simulink model "flightControlSystem"  (R2026a)
settings: Solver=ode3  StartTime=0  StopTime=TFinal  FixedStep=Ts  EnableMultiTasking=on
undefined symbols (not defined in the file): codertarget, Controller, DiscIntNeverNeededParam, Discrete, Estimator, g, gray, init, Sensors, Time, Ts, var_acc_angle_N, var_bias_gyr_N, var_gyro_p_N, Vehicle
libraries: simulink x39, slpidlib x4, ctrlSharedLib x4, sharedtransform x3, parrotlib x1
(part 2 of 2)

== system flightControlSystem/Control System/Crash Predictor Flags/Normal condition ==
  Action Port : ActionPort  ActionPortLabel=else
  Constant : Constant  Value=0  OutDataTypeStr=uint8
  Out1 : Outport  VectorParamsAs1DForOutWhenUnconnected=off
  wires:
  Constant/1 -> Out1/1

== system flightControlSystem/Control System/Crash Predictor Flags/Ultrasound improper ==
  Action Port : ActionPort  ActionPortLabel=elseif(u4>0)
  Constant : Constant  Value=0  OutDataTypeStr=uint8
  Out1 : Outport  VectorParamsAs1DForOutWhenUnconnected=off
  wires:
  Constant/1 -> Out1/1

== system flightControlSystem/Control System/Crash Predictor Flags/estimator//Optical flow error ==
  Action Port : ActionPort  ActionPortLabel=elseif(u2 > 0)
  Constant : Constant  Value=99  OutDataTypeStr=uint8
  Out1 : Outport  VectorParamsAs1DForOutWhenUnconnected=off
  wires:
  Constant/1 -> Out1/1

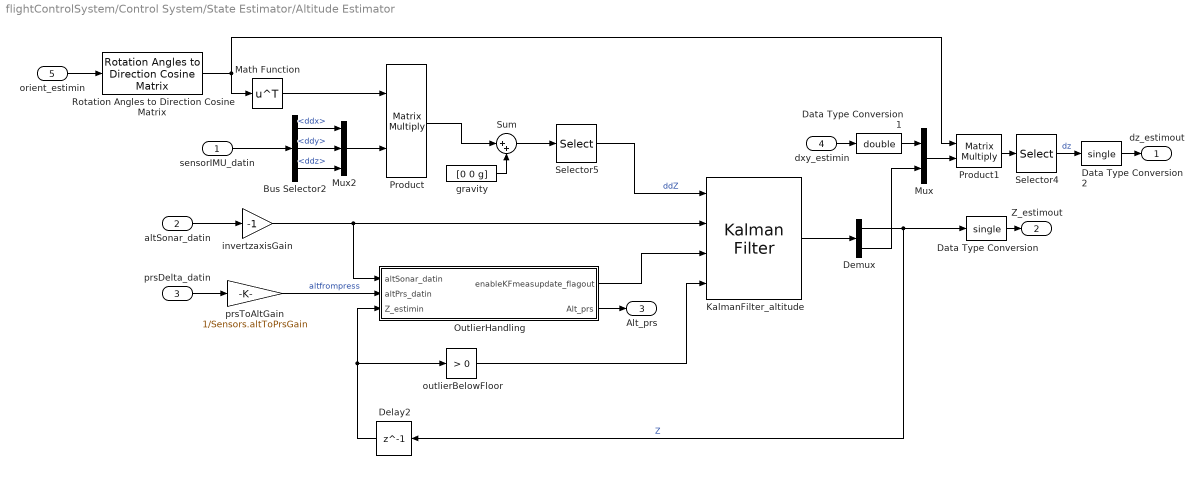
== system flightControlSystem/Control System/State Estimator/Altitude Estimator ==
  sensorIMU_datin : Inport
  altSonar_datin : Inport  Port=2
  prsDelta_datin : Inport  Port=3
  dxy_estimin : Inport  Port=4
  orient_estimin : Inport  Port=5
  Bus Selector2 : BusSelector  OutputSignals=ddx,ddy,ddz
  Data Type Conversion : DataTypeConversion  OutDataTypeStr=single  RndMeth=Floor
  Data Type Conversion1 : DataTypeConversion  OutDataTypeStr=double  RndMeth=Floor
  Data Type Conversion2 : DataTypeConversion  OutDataTypeStr=single  RndMeth=Floor
  Delay2 : Delay  DelayLength=1  InitialCondition=0
  Demux : Demux  Outputs=2
  KalmanFilter_altitude : ctrlSharedLib/Kalman Filter  TimeDomain=Discrete-Time  UseCurrentEstimator=on  ModelSource=Individual A, B, C, D matrices  ModelSourceVariable=sys  A=[1 Ts; 0 1]  B=[0;Ts]  C=[1 0]  D=[0]  NumberOfStates=2  NumberOfInputs=2  NumberOfOutputs=2  Ts=-1  InitialEstimateSource=Dialog  X0=[init.posNED(3) 0]  P0=10  UseK=off  UseGH=on  G=Estimator.alt.kf.G  TimeInvariantG=on  H=Estimator.alt.kf.H  TimeInvariantH=on  NumberOfProcessNoiseInputs=2  Q=Estimator.alt.kf.Q  TimeInvariantQ=on  R=Estimator.alt.kf.R  TimeInvariantR=on  N=Estimator.alt.kf.N  TimeInvariantN=on  AddInputPort=on  AddEnablePort=on  ExternalReset=Level hold  OutputEstimatedY=off  OutputP=off
  Math Function : Math  Operator=transpose  SignedPower=on
  Mux : Mux  Inputs=2
  Mux2 : Mux  Inputs=3
  OutlierHandling : Subsystem
  Product : Product  Multiplication=Matrix(*)
  Product1 : Product  Multiplication=Matrix(*)
  Rotation Angles to Direction Cosine Matrix : sharedtransform/Rotation Angles to Direction Cosine Matrix  rotationOrder=ZYX  aMode=aMode
  Selector4 : Selector  InputPortWidth=3  IndexOptions=Index vector (dialog)  Indices=[3]  OutputSizes=1
  Selector5 : Selector  InputPortWidth=3  IndexOptions=Index vector (dialog)  Indices=[3]  OutputSizes=1
  Sum : Sum  Inputs=|++
  gravity : Constant  Value=[0 0 g]
  invertzaxisGain : Gain  Gain=-1  ParamDataTypeStr=single  OutDataTypeStr=double
  outlierBelowFloor : simulink/Logic and Bit Operations/Compare To Constant  relop=>  const=0  OutDataTypeStr=boolean
  prsToAltGain : Gain  Gain=1/Sensors.altToPrsGain
  dz_estimout : Outport  VectorParamsAs1DForOutWhenUnconnected=off
  Z_estimout : Outport  Port=2  VectorParamsAs1DForOutWhenUnconnected=off
  Alt_prs : Outport  Port=3  VectorParamsAs1DForOutWhenUnconnected=off
  wires:
  Mux2/1 -> Product/2
  sensorIMU_datin/1 -> Bus Selector2/1
  Bus Selector2/3 -> Mux2/3  "<ddz>"
  Bus Selector2/2 -> Mux2/2  "<ddy>"
  Bus Selector2/1 -> Mux2/1  "<ddx>"
  Product1/1 -> Selector4/1
  dxy_estimin/1 -> Data Type Conversion1/1
  Delay2/1 -> OutlierHandling/3(Z_estimin), outlierBelowFloor/1
  prsToAltGain/1 -> OutlierHandling/2(altPrs_datin)  "altfrompress"
  prsDelta_datin/1 -> prsToAltGain/1
  outlierBelowFloor/1 -> KalmanFilter_altitude/4
  Demux/2 -> Mux/2
  Selector4/1 -> Data Type Conversion2/1  "dz"
  Demux/1 -> Data Type Conversion/1, Delay2/1  "Z"
  Selector5/1 -> KalmanFilter_altitude/1  "ddZ"
  Mux/1 -> Product1/2
  KalmanFilter_altitude/1 -> Demux/1
  Sum/1 -> Selector5/1
  gravity/1 -> Sum/2
  Product/1 -> Sum/1
  altSonar_datin/1 -> invertzaxisGain/1
  orient_estimin/1 -> Rotation Angles to Direction Cosine Matrix/1
  Data Type Conversion/1 -> Z_estimout/1
  Data Type Conversion1/1 -> Mux/1
  Math Function/1 -> Product/1
  invertzaxisGain/1 -> KalmanFilter_altitude/2, OutlierHandling/1(altSonar_datin)
  Data Type Conversion2/1 -> dz_estimout/1
  OutlierHandling/1(enableKFmeasupdate_flagout) -> KalmanFilter_altitude/3
  Rotation Angles to Direction Cosine Matrix/1 -> Math Function/1, Product1/1
  OutlierHandling/2(Alt_prs) -> Alt_prs/1

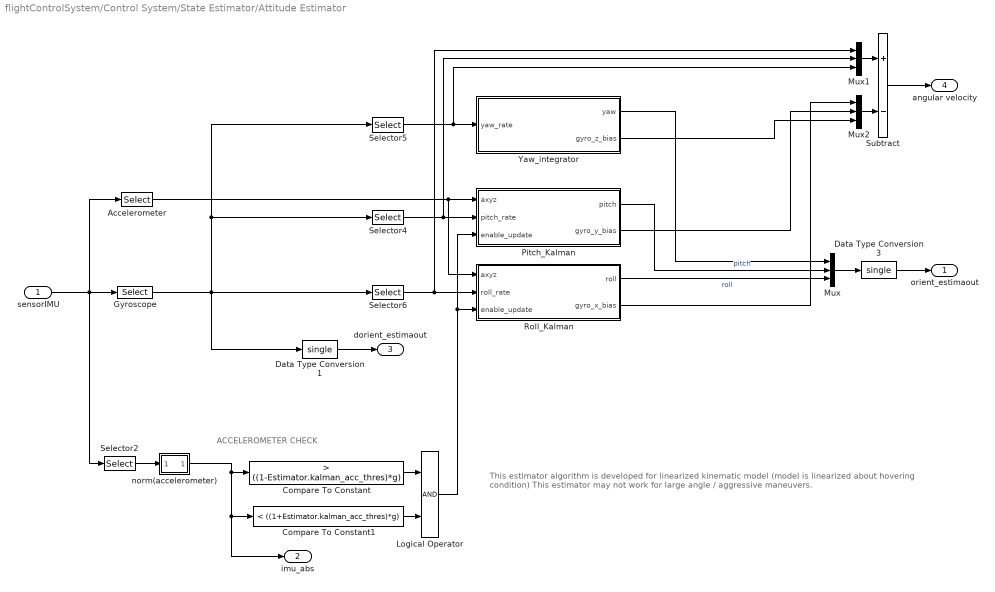
== system flightControlSystem/Control System/State Estimator/Attitude Estimator ==
  note: ACCELEROMETER CHECK
  note: This estimator algorithm is developed for linearized kinematic model (model is linearized about hovering condition)
      | This estimator may not work for large angle / aggressive maneuvers.
  sensorIMU : Inport  OutDataTypeStr=single
  Accelerometer : Selector  InputPortWidth=6  IndexOptions=Index vector (dialog)  Indices=[1 2 3]  OutputSizes=1
  Compare To Constant : simulink/Logic and Bit Operations/Compare To Constant  relop=>  const=((1-Estimator.kalman_acc_thres)*g)  OutDataTypeStr=boolean
  Compare To Constant1 : simulink/Logic and Bit Operations/Compare To Constant  relop=<  const=((1+Estimator.kalman_acc_thres)*g)  OutDataTypeStr=boolean
  Data Type Conversion1 : DataTypeConversion  OutDataTypeStr=single  SaturateOnIntegerOverflow=off  RndMeth=Floor
  Data Type Conversion3 : DataTypeConversion  OutDataTypeStr=single  SaturateOnIntegerOverflow=off  RndMeth=Floor
  Gyroscope : Selector  InputPortWidth=6  IndexOptions=Index vector (dialog)  Indices=[4 5 6]  OutputSizes=1
  Logical Operator : Logic  AllPortsSameDT=off  OutDataTypeStr=fixdt(1,16)
  Mux : Mux  Inputs=3
  Mux1 : Mux  Inputs=3
  Mux2 : Mux  Inputs=3
  Pitch_Kalman : Subsystem
  Roll_Kalman : Subsystem
  Selector2 : Selector  InputPortWidth=6  IndexOptions=Index vector (dialog)  Indices=[1 2 3]  OutputSizes=1
  Selector4 : Selector  InputPortWidth=3  IndexOptions=Index vector (dialog)  Indices=[2]  OutputSizes=1
  Selector5 : Selector  InputPortWidth=3  IndexOptions=Index vector (dialog)  Indices=[3]  OutputSizes=1
  Selector6 : Selector  InputPortWidth=3  IndexOptions=Index vector (dialog)  Indices=[1]  OutputSizes=1
  Subtract : Sum  Inputs=+-
  Yaw_integrator : Subsystem
  norm(accelerometer) : Subsystem
  orient_estimaout : Outport  VectorParamsAs1DForOutWhenUnconnected=off
  imu_abs : Outport  Port=2  OutDataTypeStr=single  VectorParamsAs1DForOutWhenUnconnected=off
  dorient_estimaout : Outport  Port=3  VectorParamsAs1DForOutWhenUnconnected=off
  angular velocity : Outport  Port=4  VectorParamsAs1DForOutWhenUnconnected=off
  wires:
  sensorIMU/1 -> Selector2/1, Accelerometer/1, Gyroscope/1
  Compare To Constant/1 -> Logical Operator/1
  Compare To Constant1/1 -> Logical Operator/2
  Mux/1 -> Data Type Conversion3/1
  Gyroscope/1 -> Data Type Conversion1/1, Selector5/1, Selector4/1, Selector6/1
  Data Type Conversion3/1 -> orient_estimaout/1
  Data Type Conversion1/1 -> dorient_estimaout/1
  Accelerometer/1 -> Roll_Kalman/1(axyz), Pitch_Kalman/1(axyz)
  Selector4/1 -> Mux1/2, Pitch_Kalman/2(pitch_rate)
  Selector5/1 -> Mux1/3, Yaw_integrator/1(yaw_rate)
  Selector6/1 -> Mux1/1, Roll_Kalman/2(roll_rate)
  Yaw_integrator/1(yaw) -> Mux/1
  Pitch_Kalman/1(pitch) -> Mux/2  "pitch"
  Roll_Kalman/1(roll) -> Mux/3  "roll"
  Logical Operator/1 -> Roll_Kalman/3(enable_update), Pitch_Kalman/3(enable_update)
  Mux1/1 -> Subtract/1
  Subtract/1 -> angular velocity/1
  Roll_Kalman/2(gyro_x_bias) -> Mux2/1
  Pitch_Kalman/2(gyro_y_bias) -> Mux2/2
  Yaw_integrator/2(gyro_z_bias) -> Mux2/3
  Mux2/1 -> Subtract/2
  norm(accelerometer)/1(Out1) -> imu_abs/1, Compare To Constant1/1, Compare To Constant/1
  Selector2/1 -> norm(accelerometer)/1(In1)

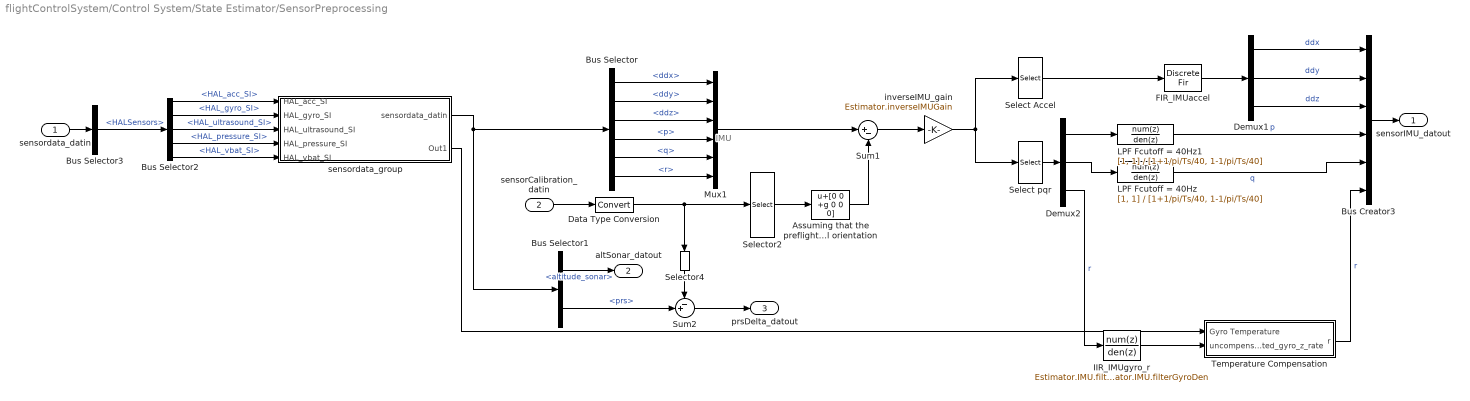
== system flightControlSystem/Control System/State Estimator/SensorPreprocessing ==
  note: IMU
  sensordata_datin : Inport
  sensorCalibration_datin : Inport  Port=2
  Assuming that the preflight calibration was done at level orientation : Bias  Bias=[0 0 +g 0 0 0]  SaturateOnIntegerOverflow=off
  Bus Creator3 : BusCreator  Inputs=6
  Bus Selector : BusSelector  OutputSignals=ddx,ddy,ddz,p,q,r
  Bus Selector1 : BusSelector  OutputSignals=altitude_sonar,prs
  Bus Selector2 : BusSelector  OutputSignals=HAL_acc_SI,HAL_gyro_SI,HAL_ultrasound_SI,HAL_pressure_SI,HAL_vbat_SI
  Bus Selector3 : BusSelector  OutputSignals=HALSensors
  Data Type Conversion : DataTypeConversion  SaturateOnIntegerOverflow=off  RndMeth=Floor
  Demux1 : Demux  Outputs=3
  Demux2 : Demux  Outputs=3
  FIR_IMUaccel : DiscreteFir  Coefficients=Estimator.IMU.filterAccel.Coefficients
  IIR_IMUgyro_r : DiscreteFilter  Numerator=Estimator.IMU.filterGyroNum  Denominator=Estimator.IMU.filterGyroDen
  LPF Fcutoff = 40Hz : DiscreteTransferFcn  Numerator=[1, 1]  Denominator=[1+1/pi/Ts/40, 1-1/pi/Ts/40]
  LPF Fcutoff = 40Hz1 : DiscreteTransferFcn  Numerator=[1, 1]  Denominator=[1+1/pi/Ts/40, 1-1/pi/Ts/40]
  Mux1 : Mux  Inputs=6
  Select Accel : Selector  InputPortWidth=6  IndexOptions=Index vector (dialog)  Indices=[1 2 3]  OutputSizes=1
  Select pqr : Selector  InputPortWidth=6  IndexOptions=Index vector (dialog)  Indices=[4 5 6]  OutputSizes=1
  Selector2 : Selector  InputPortWidth=8  IndexOptions=Index vector (dialog)  Indices=[1:6]  OutputSizes=1
  Selector4 : Selector  InputPortWidth=8  IndexOptions=Index vector (dialog)  Indices=[7]  OutputSizes=1
  Sum1 : Sum  Inputs=|+-
  Sum2 : Sum  Inputs=-+|
  Temperature Compensation : Subsystem
  inverseIMU_gain : Gain  Gain=Estimator.inverseIMUGain  ParamDataTypeStr=single  OutDataTypeStr=single
  sensordata_group : Subsystem
  sensorIMU_datout : Outport  VectorParamsAs1DForOutWhenUnconnected=off
  altSonar_datout : Outport  Port=2  VectorParamsAs1DForOutWhenUnconnected=off
  prsDelta_datout : Outport  Port=3  VectorParamsAs1DForOutWhenUnconnected=off
  wires:
  Select pqr/1 -> Demux2/1
  Assuming that the preflight calibration was done at level orientation/1 -> Sum1/2
  Mux1/1 -> Sum1/1
  Sum2/1 -> prsDelta_datout/1
  Bus Selector1/2 -> Sum2/2  "<prs>"
  Selector4/1 -> Sum2/1
  Bus Selector1/1 -> altSonar_datout/1  "<altitude_sonar>"
  Bus Selector/6 -> Mux1/6  "<r>"
  Bus Selector/5 -> Mux1/5  "<q>"
  Bus Selector/4 -> Mux1/4  "<p>"
  Bus Selector/3 -> Mux1/3  "<ddz>"
  Bus Selector/2 -> Mux1/2  "<ddy>"
  Bus Selector/1 -> Mux1/1  "<ddx>"
  sensorCalibration_datin/1 -> Data Type Conversion/1
  Demux2/3 -> IIR_IMUgyro_r/1  "r"
  FIR_IMUaccel/1 -> Demux1/1
  Select Accel/1 -> FIR_IMUaccel/1
  inverseIMU_gain/1 -> Select Accel/1, Select pqr/1
  Demux2/2 -> LPF Fcutoff = 40Hz/1
  Demux2/1 -> LPF Fcutoff = 40Hz1/1
  Selector2/1 -> Assuming that the preflight calibration was done at level orientation/1
  Sum1/1 -> inverseIMU_gain/1
  Demux1/3 -> Bus Creator3/3  "ddz"
  Demux1/2 -> Bus Creator3/2  "ddy"
  Demux1/1 -> Bus Creator3/1  "ddx"
  Bus Creator3/1 -> sensorIMU_datout/1
  Data Type Conversion/1 -> Selector2/1, Selector4/1
  Bus Selector2/2 -> sensordata_group/2(HAL_gyro_SI)  "<HAL_gyro_SI>"
  Bus Selector2/4 -> sensordata_group/4(HAL_pressure_SI)  "<HAL_pressure_SI>"
  Bus Selector2/5 -> sensordata_group/5(HAL_vbat_SI)  "<HAL_vbat_SI>"
  Bus Selector2/3 -> sensordata_group/3(HAL_ultrasound_SI)  "<HAL_ultrasound_SI>"
  Bus Selector3/1 -> Bus Selector2/1  "<HALSensors>"
  sensordata_group/1(sensordata_datin) -> Bus Selector1/1, Bus Selector/1
  sensordata_datin/1 -> Bus Selector3/1
  Bus Selector2/1 -> sensordata_group/1(HAL_acc_SI)  "<HAL_acc_SI>"
  LPF Fcutoff = 40Hz1/1 -> Bus Creator3/4  "p"
  LPF Fcutoff = 40Hz/1 -> Bus Creator3/5  "q"
  sensordata_group/2(Out1) -> Temperature Compensation/1(Gyro Temperature)
  IIR_IMUgyro_r/1 -> Temperature Compensation/2(uncompensated_gyro_z_rate)
  Temperature Compensation/1(r) -> Bus Creator3/6  "r"

== system flightControlSystem/Control System/State Estimator/XY Position Estimator ==
  opticalFlow_datin : Inport
  controlModePosVSOrient_flagin : Inport  Port=2
  sensorIMU_datin : Inport  Port=3
  Z_estimin : Inport  Port=4
  dz_estimin : Inport  Port=5
  orient_estimin : Inport  Port=6
  Angular velocity : Inport  Port=7
  EstimatorVelocity : Subsystem
  EstimatorXYPosition : Subsystem
  XY_estimout : Outport  VectorParamsAs1DForOutWhenUnconnected=off
  dxy_estimout : Outport  Port=2  VectorParamsAs1DForOutWhenUnconnected=off
  wires:
  EstimatorXYPosition/1(XY_estimout) -> XY_estimout/1
  dz_estimin/1 -> EstimatorXYPosition/4(dz_estimin)
  controlModePosVSOrient_flagin/1 -> EstimatorXYPosition/3(controlModePosVSOrient_flagin)
  Z_estimin/1 -> EstimatorVelocity/2(Z_estimin)
  sensorIMU_datin/1 -> EstimatorVelocity/3(sensorIMU_datin)
  opticalFlow_datin/1 -> EstimatorVelocity/1(opticalFlow_datin)
  EstimatorVelocity/1(dxy_estimout) -> dxy_estimout/1, EstimatorXYPosition/1(dxy_estimin)
  orient_estimin/1 -> EstimatorXYPosition/2(orient_estimin), EstimatorVelocity/4(orient_estimin)
  Angular velocity/1 -> EstimatorVelocity/5(angular velocity)

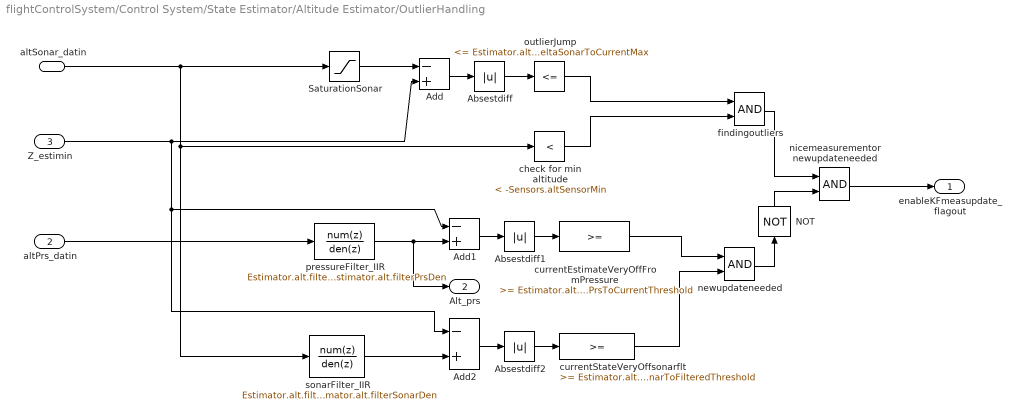
== system flightControlSystem/Control System/State Estimator/Altitude Estimator/OutlierHandling ==
  altSonar_datin : Inport
  altPrs_datin : Inport  Port=2
  Z_estimin : Inport  Port=3
  Absestdiff : Abs  SaturateOnIntegerOverflow=off
  Absestdiff1 : Abs  SaturateOnIntegerOverflow=off
  Absestdiff2 : Abs  SaturateOnIntegerOverflow=off
  Add : Sum  Inputs=-+
  Add1 : Sum  Inputs=-+
  Add2 : Sum  Inputs=-+
  NOT : Logic  Operator=NOT  IconShape=distinctive  AllPortsSameDT=off  OutDataTypeStr=boolean
  SaturationSonar : Saturate  UpperLimit=-Sensors.altSensorMin  LowerLimit=-inf
  check for min altitude : simulink/Logic and Bit Operations/Compare To Constant  relop=<  const=-Sensors.altSensorMin  OutDataTypeStr=boolean
  currentEstimateVeryOffFromPressure : simulink/Logic and Bit Operations/Compare To Constant  relop=>=  const=Estimator.alt.deltaPrsToCurrentThreshold  OutDataTypeStr=boolean
  currentStateVeryOffsonarflt : simulink/Logic and Bit Operations/Compare To Constant  relop=>=  const=Estimator.alt.deltaSonarToFilteredThreshold  OutDataTypeStr=boolean
  findingoutliers : Logic  AllPortsSameDT=off  OutDataTypeStr=boolean
  newupdateneeded : Logic  AllPortsSameDT=off  OutDataTypeStr=boolean
  nicemeasurementor newupdateneeded : Logic  AllPortsSameDT=off  OutDataTypeStr=boolean
  outlierJump : simulink/Logic and Bit Operations/Compare To Constant  relop=<=  const=Estimator.alt.deltaSonarToCurrentMax  OutDataTypeStr=boolean
  pressureFilter_IIR : DiscreteFilter  Numerator=Estimator.alt.filterPrsNum  Denominator=Estimator.alt.filterPrsDen
  sonarFilter_IIR : DiscreteFilter  Numerator=Estimator.alt.filterSonarNum  Denominator=Estimator.alt.filterSonarDen
  enableKFmeasupdate_flagout : Outport  VectorParamsAs1DForOutWhenUnconnected=off
  Alt_prs : Outport  Port=2  VectorParamsAs1DForOutWhenUnconnected=off
  wires:
  Add1/1 -> Absestdiff1/1
  nicemeasurementor newupdateneeded/1 -> enableKFmeasupdate_flagout/1
  findingoutliers/1 -> nicemeasurementor newupdateneeded/1
  check for min altitude/1 -> findingoutliers/2
  outlierJump/1 -> findingoutliers/1
  SaturationSonar/1 -> Add/1
  Absestdiff/1 -> outlierJump/1
  Add/1 -> Absestdiff/1
  newupdateneeded/1 -> NOT/1
  Absestdiff2/1 -> currentStateVeryOffsonarflt/1
  altSonar_datin/1 -> SaturationSonar/1, sonarFilter_IIR/1, check for min altitude/1
  currentEstimateVeryOffFromPressure/1 -> newupdateneeded/1
  Z_estimin/1 -> Add1/1, Add2/1, Add/2
  Add2/1 -> Absestdiff2/1
  currentStateVeryOffsonarflt/1 -> newupdateneeded/2
  pressureFilter_IIR/1 -> Alt_prs/1, Add1/2
  altPrs_datin/1 -> pressureFilter_IIR/1
  sonarFilter_IIR/1 -> Add2/2
  Absestdiff1/1 -> currentEstimateVeryOffFromPressure/1
  NOT/1 -> nicemeasurementor newupdateneeded/2

== system flightControlSystem/Control System/State Estimator/Attitude Estimator/Pitch_Kalman ==
  note: Gyroscope's bias is susceptible to factors like "temperature" and "Gyro bias stability" and it
      | can vary during the flight. It is therefore estimated using this Kalman filter making use of Accelerometer data
  note: Linear Kalman filter is used for the Pitch and Roll estimation.
      | The states are the corresponding Euler angle and Angular rate bias respectively
  axyz : Inport
  pitch_rate : Inport  Port=2
  enable_update : Inport  Port=3
  Demux : Demux  Outputs=2
  Gain2 : Gain  Gain=1/g
  Kalman Filter : ctrlSharedLib/Kalman Filter  TimeDomain=Discrete-Time  UseCurrentEstimator=on  ModelSource=Individual A, B, C, D matrices  ModelSourceVariable=ss(0.95,1,1,0,1)  A=[1 -Ts;0 1]  B=[Ts;0]  C=[1 0]  D=0  NumberOfStates=1  NumberOfInputs=1  NumberOfOutputs=1  Ts=Ts  InitialEstimateSource=Dialog  X0=0  P0=10  UseK=off  UseGH=off  G=1  TimeInvariantG=on  H=0  TimeInvariantH=on  NumberOfProcessNoiseInputs=1  Q=[var_gyro_p_N,0;0,var_bias_gyr_N]  TimeInvariantQ=on  R=var_acc_angle_N  TimeInvariantR=on  N=0  TimeInvariantN=on  AddInputPort=on  AddEnablePort=on  OutputEstimatedY=off  OutputP=off
  Selector1 : Selector  InputPortWidth=3  IndexOptions=Index vector (dialog)  Indices=[1]  OutputSizes=1
  Trigonometric Function1 : Trigonometry  Operator=asin
  single : DataTypeConversion  OutDataTypeStr=single  SaturateOnIntegerOverflow=off  RndMeth=Floor
  single1 : DataTypeConversion  OutDataTypeStr=single  SaturateOnIntegerOverflow=off  RndMeth=Floor
  pitch : Outport
  gyro_y_bias : Outport  Port=2
  wires:
  Kalman Filter/1 -> Demux/1
  Demux/1 -> single1/1
  Gain2/1 -> Trigonometric Function1/1
  Trigonometric Function1/1 -> Kalman Filter/2
  Selector1/1 -> Gain2/1
  axyz/1 -> Selector1/1
  pitch_rate/1 -> Kalman Filter/1
  enable_update/1 -> Kalman Filter/3
  Demux/2 -> single/1
  single/1 -> gyro_y_bias/1
  single1/1 -> pitch/1

== system flightControlSystem/Control System/State Estimator/Attitude Estimator/Roll_Kalman ==
  note: Linear Kalman filter is used for the Pitch and Roll estimation.
      | The states are the corresponding Euler angle and Angular rate bias respectively
  note: Gyroscope's bias is susceptible to factors like "temperature" and "Gyro bias stability" and it
      | can vary during the flight. It is therefore estimated using the Kalman filter making use of accelerometer data
  axyz : Inport
  roll_rate : Inport  Port=2
  enable_update : Inport  Port=3
  Data Type Conversion : DataTypeConversion  SaturateOnIntegerOverflow=off  RndMeth=Floor
  Data Type Conversion1 : DataTypeConversion  SaturateOnIntegerOverflow=off  RndMeth=Floor
  Demux : Demux  Outputs=3
  Demux1 : Demux  Outputs=2
  Divide : Product  Inputs=*/
  Kalman Filter : ctrlSharedLib/Kalman Filter  TimeDomain=Discrete-Time  UseCurrentEstimator=on  ModelSource=Individual A, B, C, D matrices  ModelSourceVariable=ss(0.95,1,1,0,1)  A=[1 -Ts;0 1]  B=[Ts;0]  C=[1 0]  D=0  NumberOfStates=1  NumberOfInputs=1  NumberOfOutputs=1  Ts=Ts  InitialEstimateSource=Dialog  X0=0  P0=10  UseK=off  UseGH=off  G=1  TimeInvariantG=on  H=0  TimeInvariantH=on  NumberOfProcessNoiseInputs=1  Q=[var_gyro_p_N,0;0,var_bias_gyr_N]  TimeInvariantQ=on  R=var_acc_angle_N  TimeInvariantR=on  N=0  TimeInvariantN=on  AddInputPort=on  AddEnablePort=on  OutputEstimatedY=off  OutputP=off
  Terminator : Terminator
  Trigonometric Function : Trigonometry  Operator=atan
  roll : Outport
  gyro_x_bias : Outport  Port=2
  wires:
  Demux1/1 -> Data Type Conversion1/1
  Kalman Filter/1 -> Demux1/1
  roll_rate/1 -> Kalman Filter/1
  Divide/1 -> Trigonometric Function/1
  Demux/2 -> Divide/1
  axyz/1 -> Demux/1
  Demux/3 -> Divide/2
  Trigonometric Function/1 -> Kalman Filter/2
  enable_update/1 -> Kalman Filter/3
  Demux1/2 -> Data Type Conversion/1
  Data Type Conversion/1 -> gyro_x_bias/1
  Data Type Conversion1/1 -> roll/1
  Demux/1 -> Terminator/1

== system flightControlSystem/Control System/State Estimator/Attitude Estimator/Yaw_integrator ==
  note: Yaw angle is not constrained between -180 to 180 degrees
  note: Currently yaw angle is obtained solely by integrating the gyroscope output.
      | This yaw estimate can drift with time.
  yaw_rate : Inport
  Constant : Constant  Value=0  OutDataTypeStr=single
  Discrete-Time Integrator : DiscreteIntegrator  SampleTime=-1  ICPrevOutput=DiscIntNeverNeededParam  ICPrevScaledInput=DiscIntNeverNeededParam
  yaw : Outport
  gyro_z_bias : Outport  Port=2
  wires:
  yaw_rate/1 -> Discrete-Time Integrator/1
  Discrete-Time Integrator/1 -> yaw/1
  Constant/1 -> gyro_z_bias/1

== system flightControlSystem/Control System/State Estimator/Attitude Estimator/norm(accelerometer) ==
  In1 : Inport
  Constant : Constant  Value=2  OutDataTypeStr=single
  Data Type Conversion2 : DataTypeConversion  OutDataTypeStr=single  SaturateOnIntegerOverflow=off  RndMeth=Floor
  Math Function : Math  Operator=pow  SignedPower=on
  Sqrt : Sqrt
  Sum of Elements : Sum  Inputs=+
  Out1 : Outport
  wires:
  Sum of Elements/1 -> Sqrt/1
  Math Function/1 -> Sum of Elements/1
  Data Type Conversion2/1 -> Math Function/1
  In1/1 -> Data Type Conversion2/1
  Constant/1 -> Math Function/2
  Sqrt/1 -> Out1/1

== system flightControlSystem/Control System/State Estimator/SensorPreprocessing/Temperature Compensation ==
  note: Gyroscope's bias is affected by temperature.This won't be a problem for Pitch and Roll angle estimation as the actual gyroscope bias in the Pitch and Roll axis are estimated during the flight. However the yaw orientation is obtained by integrating the gyroscope output and it may drift with time. Even the preflight calibration which is done cannot compensate for this problem as the gyro bis varies during the flight.
  Gyro Temperature : Inport
  uncompensated_gyro_z_rate : Inport  Port=2
  Compare To Constant : simulink/Logic and Bit Operations/Compare To Constant  relop===  const=1  OutDataTypeStr=boolean
  Constant : Constant  Value=0
  Counter Free-Running : simulink/Sources/Counter Free-Running  NumBits=32  tsamp=0.005
  Data Type Conversion1 : DataTypeConversion  SaturateOnIntegerOverflow=off  RndMeth=Floor
  Disable temperature compensation : ManualSwitch
  Gain : Gain  Gain=0.00228
  Subtract : Sum  Inputs=+-
  Subtract1 : Sum  Inputs=+-
  Triggered Subsystem : Subsystem  TreatAsAtomicUnit=on
  r : Outport
  wires:
  Gain/1 -> Disable temperature compensation/1
  Disable temperature compensation/1 -> Data Type Conversion1/1
  Gyro Temperature/1 -> Subtract/1, Triggered Subsystem/1(In1)
  Triggered Subsystem/1(Out1) -> Subtract/2  "Initial temperature"
  Compare To Constant/1 -> Triggered Subsystem/Trigger
  Constant/1 -> Disable temperature compensation/2
  Subtract/1 -> Gain/1
  Data Type Conversion1/1 -> Subtract1/2
  Counter Free-Running/1 -> Compare To Constant/1
  uncompensated_gyro_z_rate/1 -> Subtract1/1
  Subtract1/1 -> r/1  "r"

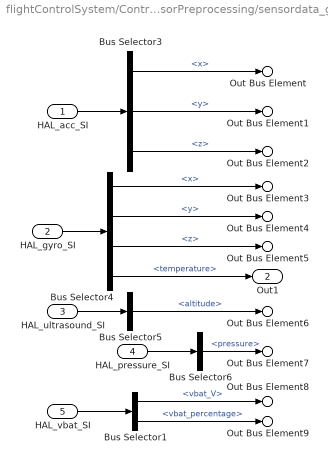
== system flightControlSystem/Control System/State Estimator/SensorPreprocessing/sensordata_group ==
  HAL_acc_SI : Inport  OutDataTypeStr=Bus: HAL_acc_SI_t
  HAL_gyro_SI : Inport  Port=2  OutDataTypeStr=Bus: HAL_gyro_SI_t
  HAL_ultrasound_SI : Inport  Port=3  OutDataTypeStr=Bus: HAL_ultrasound_SI_t
  HAL_pressure_SI : Inport  Port=4  OutDataTypeStr=Bus: HAL_pressure_SI_t
  HAL_vbat_SI : Inport  Port=5  OutDataTypeStr=Bus: HAL_vbat_SI_t
  Bus Selector1 : BusSelector  OutputSignals=vbat_V,vbat_percentage
  Bus Selector3 : BusSelector  OutputSignals=x,y,z
  Bus Selector4 : BusSelector  OutputSignals=x,y,z,temperature
  Bus Selector5 : BusSelector  OutputSignals=altitude
  Bus Selector6 : BusSelector  OutputSignals=pressure
  Out Bus Element : Outport  VectorParamsAs1DForOutWhenUnconnected=off  PortName=sensordata_datin  Element=ddx
  Out Bus Element1 : Outport  VectorParamsAs1DForOutWhenUnconnected=off  PortName=sensordata_datin  Element=ddy
  Out Bus Element2 : Outport  VectorParamsAs1DForOutWhenUnconnected=off  PortName=sensordata_datin  Element=ddz
  Out Bus Element3 : Outport  VectorParamsAs1DForOutWhenUnconnected=off  PortName=sensordata_datin  Element=p
  Out Bus Element4 : Outport  VectorParamsAs1DForOutWhenUnconnected=off  PortName=sensordata_datin  Element=q
  Out Bus Element5 : Outport  VectorParamsAs1DForOutWhenUnconnected=off  PortName=sensordata_datin  Element=r
  Out Bus Element6 : Outport  VectorParamsAs1DForOutWhenUnconnected=off  PortName=sensordata_datin  Element=altitude_sonar
  Out Bus Element7 : Outport  VectorParamsAs1DForOutWhenUnconnected=off  PortName=sensordata_datin  Element=prs
  Out Bus Element8 : Outport  VectorParamsAs1DForOutWhenUnconnected=off  PortName=sensordata_datin  Element=vbat_V
  Out Bus Element9 : Outport  VectorParamsAs1DForOutWhenUnconnected=off  PortName=sensordata_datin  Element=vbat_percentage
  Out1 : Outport  Port=2
  wires:
  HAL_gyro_SI/1 -> Bus Selector4/1
  HAL_acc_SI/1 -> Bus Selector3/1
  HAL_pressure_SI/1 -> Bus Selector6/1
  HAL_ultrasound_SI/1 -> Bus Selector5/1
  Bus Selector4/1 -> Out Bus Element3/1  "<x>"
  Bus Selector3/3 -> Out Bus Element2/1  "<z>"
  Bus Selector4/3 -> Out Bus Element5/1  "<z>"
  Bus Selector5/1 -> Out Bus Element6/1  "<altitude>"
  Bus Selector6/1 -> Out Bus Element7/1  "<pressure>"
  Bus Selector4/2 -> Out Bus Element4/1  "<y>"
  Bus Selector3/1 -> Out Bus Element/1  "<x>"
  Bus Selector3/2 -> Out Bus Element1/1  "<y>"
  Bus Selector1/1 -> Out Bus Element8/1  "<vbat_V>"
  HAL_vbat_SI/1 -> Bus Selector1/1
  Bus Selector1/2 -> Out Bus Element9/1  "<vbat_percentage>"
  Bus Selector4/4 -> Out1/1  "<temperature>"

== system flightControlSystem/Control System/State Estimator/XY Position Estimator/EstimatorVelocity ==
  opticalFlow_datin : Inport
  Z_estimin : Inport  Port=2  SampleTime=Ts
  sensorIMU_datin : Inport  Port=3
  orient_estimin : Inport  Port=4
  angular velocity : Inport  Port=5
  AccelerationHandling : Subsystem
  Angular velocity compensation for optical flow : Subsystem
  DataHandling : Subsystem
  Delay : Delay  DelayLength=1  InitialCondition=0
  KalmanFilter_dxdy : ctrlSharedLib/Kalman Filter  TimeDomain=Discrete-Time  UseCurrentEstimator=on  ModelSource=Individual A, B, C, D matrices  ModelSourceVariable=ss(0.95,1,1,0,1)  A=Estimator.pos.kfVelo.A  B=Estimator.pos.kfVelo.B  C=Estimator.pos.kfVelo.C  D=Estimator.pos.kfVelo.D  NumberOfStates=1  NumberOfInputs=1  NumberOfOutputs=1  Ts=-1  InitialEstimateSource=Dialog  X0=0  P0=10  UseK=off  UseGH=off  G=Estimator.pos.kfVelo.G  TimeInvariantG=on  H=Estimator.pos.kfVelo.H  TimeInvariantH=on  NumberOfProcessNoiseInputs=1  Q=Estimator.pos.kfVelo.Q  TimeInvariantQ=on  R=Estimator.pos.kfVelo.R  TimeInvariantR=on  N=Estimator.pos.kfVelo.N  TimeInvariantN=on  AddInputPort=on  AddEnablePort=on  OutputEstimatedY=off  OutputP=off
  Selector1 : Selector  InputPortWidth=4  IndexOptions=Index vector (dialog)  Indices=[1 2]  OutputSizes=1
  Z_estimin1 : InportShadow  Port=2  SampleTime=Ts
  angular velocity compensation : Sum
  xy velocity w/o angular velocity compensation : Subsystem
  dxy_estimout : Outport  VectorParamsAs1DForOutWhenUnconnected=off
  wires:
  Z_estimin/1 -> DataHandling/1(Z_estimin), AccelerationHandling/4(Z_estimin)
  KalmanFilter_dxdy/1 -> Selector1/1
  sensorIMU_datin/1 -> AccelerationHandling/2(sensorIMU_datin), DataHandling/3(sensorIMU_datin)
  orient_estimin/1 -> AccelerationHandling/3(orient_estimin), DataHandling/2(orient_estimin)
  Z_estimin1/1 -> xy velocity w/o angular velocity compensation/2(z_estimate), Angular velocity compensation for optical flow/1(z_estimate)
  AccelerationHandling/1(acceleration_world) -> KalmanFilter_dxdy/1
  angular velocity compensation/1 -> KalmanFilter_dxdy/2
  Delay/1 -> DataHandling/5(dxyOF_datin)
  Selector1/1 -> dxy_estimout/1, Delay/1
  angular velocity/1 -> Angular velocity compensation for optical flow/2(Angular velocity w/o bias)
  Angular velocity compensation for optical flow/1(angular velocity correction) -> angular velocity compensation/2
  xy velocity w/o angular velocity compensation/1(optical_flow_dx_dy) -> DataHandling/4(dxy_estimin), AccelerationHandling/1(dxy_estimin), angular velocity compensation/1
  opticalFlow_datin/1 -> xy velocity w/o angular velocity compensation/1(optical_flow)
  DataHandling/1(enable_flag) -> KalmanFilter_dxdy/3

== system flightControlSystem/Control System/State Estimator/XY Position Estimator/EstimatorXYPosition ==
  note: Switching from orientationControl to Position
      | control reset the current world position estimate
      | (happens when using no markers)
  dxy_estimin : Inport
  orient_estimin : Inport  Port=2  SampleTime=Ts
  controlModePosVSOrient_flagin : Inport  Port=3
  dz_estimin : Inport  Port=4
  Math Function : Math  Operator=transpose  SignedPower=on
  Mux2 : Mux  Inputs=2
  Product : Product  Multiplication=Matrix(*)
  Rotation Angles to Direction Cosine Matrix : sharedtransform/Rotation Angles to Direction Cosine Matrix  rotationOrder=ZYX  aMode=aMode
  SelectdXY : Selector  InputPortWidth=3  IndexOptions=Index vector (dialog)  Indices=[1 2]  OutputSizes=1
  SimplyIntegrateVelocity : DiscreteIntegrator  ExternalReset=rising  SampleTime=Ts  ICPrevOutput=DiscIntNeverNeededParam  ICPrevScaledInput=DiscIntNeverNeededParam
  XY_estimout : Outport  VectorParamsAs1DForOutWhenUnconnected=off
  wires:
  controlModePosVSOrient_flagin/1 -> SimplyIntegrateVelocity/2
  Product/1 -> SelectdXY/1
  Mux2/1 -> Product/2
  dz_estimin/1 -> Mux2/2
  SimplyIntegrateVelocity/1 -> XY_estimout/1
  dxy_estimin/1 -> Mux2/1
  orient_estimin/1 -> Rotation Angles to Direction Cosine Matrix/1
  Rotation Angles to Direction Cosine Matrix/1 -> Math Function/1
  SelectdXY/1 -> SimplyIntegrateVelocity/1
  Math Function/1 -> Product/1

== system flightControlSystem/Control System/State Estimator/SensorPreprocessing/Temperature Compensation/Triggered Subsystem ==
  In1 : Inport
  Trigger : TriggerPort  TriggerType=either  VariantControl=Variant
  Out1 : Outport
  wires:
  In1/1 -> Out1/1

== system flightControlSystem/Control System/State Estimator/XY Position Estimator/EstimatorVelocity/AccelerationHandling ==
  dxy_estimin : Inport
  sensorIMU_datin : Inport  Port=2
  orient_estimin : Inport  Port=3
  Z_estimin : Inport  Port=4
  Add : Sum  Inputs=-+
  Bus Selector1 : BusSelector  OutputSignals=ddx,ddy,ddz
  Deactivate Acceleration If OF is not used due to low altitude : simulink/Logic and Bit Operations/Compare To Constant  relop=<=  const=Estimator.pos.opticalFlowZMax  OutDataTypeStr=boolean
  Logical Operator : Logic  Operator=OR  AllPortsSameDT=off  OutDataTypeStr=boolean
  Mux6 : Mux  Inputs=3
  Product : Product  Inputs=3
  Product1 : Product  Multiplication=Matrix(*)
  Rotation Angles to Direction Cosine Matrix : sharedtransform/Rotation Angles to Direction Cosine Matrix  rotationOrder=ZYX  aMode=aMode
  SelectPlanarddxy : Selector  InputPortWidth=3  IndexOptions=Index vector (dialog)  Indices=[1 2]  OutputSizes=1
  Selector : Selector  InputPortWidth=2  IndexOptions=Index vector (dialog)  Indices=1  OutputSizes=1
  Selector1 : Selector  InputPortWidth=2  IndexOptions=Index vector (dialog)  Indices=2  OutputSizes=1
  do not use acc if optical flow never available (Note OF@60Hz but ZOH to 200!) : simulink/Logic and Bit Operations/Compare To Constant  relop=~=  const=0  OutDataTypeStr=boolean
  do not use acc if optical flow never available (Note OF@60Hz but ZOH to 200!)1 : simulink/Logic and Bit Operations/Compare To Constant  relop=~=  const=0  OutDataTypeStr=boolean
  gainaccinput1 : Gain  OutDataTypeStr=single
  gravity : Constant  Value=[0 0 -g]
  acceleration_world : Outport  OutDataTypeStr=single  VectorParamsAs1DForOutWhenUnconnected=off
  wires:
  do not use acc if optical flow never available (Note OF@60Hz but ZOH to 200!)1/1 -> Logical Operator/2
  do not use acc if optical flow never available (Note OF@60Hz but ZOH to 200!)/1 -> Logical Operator/1
  Logical Operator/1 -> Product/1
  Selector1/1 -> do not use acc if optical flow never available (Note OF@60Hz but ZOH to 200!)1/1
  Selector/1 -> do not use acc if optical flow never available (Note OF@60Hz but ZOH to 200!)/1
  dxy_estimin/1 -> Selector1/1, Selector/1
  Product/1 -> acceleration_world/1
  Deactivate Acceleration If OF is not used due to low altitude/1 -> Product/3
  Z_estimin/1 -> Deactivate Acceleration If OF is not used due to low altitude/1
  Add/1 -> SelectPlanarddxy/1
  Product1/1 -> Add/1
  gravity/1 -> Product1/2
  SelectPlanarddxy/1 -> gainaccinput1/1
  Bus Selector1/3 -> Mux6/3  "<ddz>"
  Bus Selector1/1 -> Mux6/1  "<ddx>"
  sensorIMU_datin/1 -> Bus Selector1/1
  Mux6/1 -> Add/2
  Bus Selector1/2 -> Mux6/2  "<ddy>"
  orient_estimin/1 -> Rotation Angles to Direction Cosine Matrix/1
  Rotation Angles to Direction Cosine Matrix/1 -> Product1/1
  gainaccinput1/1 -> Product/2

== system flightControlSystem/Control System/State Estimator/XY Position Estimator/EstimatorVelocity/Angular velocity compensation for optical flow ==
  note: Optical flow readings are affected by both linear and angular velocity of the drone. We need to subtract the effect of angular velocity before using the flow data
  z_estimate : Inport
  Angular velocity w/o bias : Inport  Port=2
  Abs : Abs  SaturateOnIntegerOverflow=off
  Data Type Conversion : DataTypeConversion  SaturateOnIntegerOverflow=off  RndMeth=Floor
  Demux : Demux  Outputs=2
  Gain1 : Gain  Gain=-1
  Mux : Mux  Inputs=2
  Selector : Selector  InputPortWidth=3  IndexOptions=Index vector (dialog)  Indices=[1 2]  OutputSizes=1
  prod : Product  Inputs=**
  angular velocity correction : Outport
  wires:
  Gain1/1 -> Mux/1
  Mux/1 -> Data Type Conversion/1
  Demux/2 -> Gain1/1
  Data Type Conversion/1 -> angular velocity correction/1
  prod/1 -> Demux/1
  z_estimate/1 -> Abs/1
  Demux/1 -> Mux/2
  Selector/1 -> prod/2
  Abs/1 -> prod/1
  Angular velocity w/o bias/1 -> Selector/1

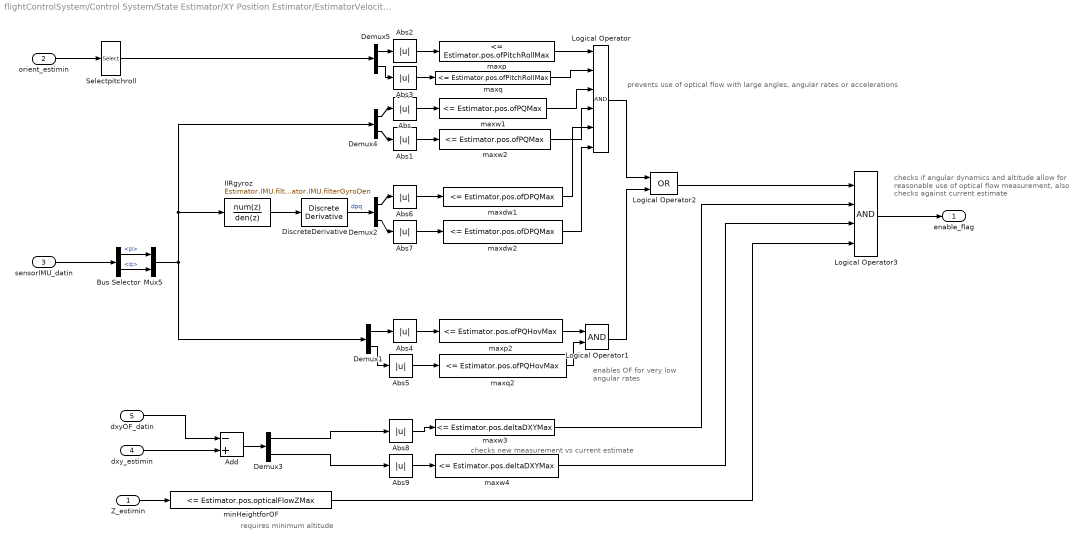
== system flightControlSystem/Control System/State Estimator/XY Position Estimator/EstimatorVelocity/DataHandling ==
  note: prevents use of optical flow with large angles, angular rates or accelerations
  note: enables OF for very
      | low angular rates
  note: checks if angular dynamics and altitude allow for
      | reasonable use of optical flow measurement,
      | also checks against current estimate
  note: checks new measurement vs current estimate
  note: requires minimum altitude
  Z_estimin : Inport
  orient_estimin : Inport  Port=2
  sensorIMU_datin : Inport  Port=3
  dxy_estimin : Inport  Port=4
  dxyOF_datin : Inport  Port=5
  Abs{,1..9} (10 alike) : Abs  SaturateOnIntegerOverflow=off
  Add : Sum  Inputs=-+
  Bus Selector : BusSelector  OutputSignals=p,q
  Demux{1..5} (5 alike) : Demux  Outputs=2
  DiscreteDerivative : simulink/Discrete/Discrete Derivative  gainval=1.0  ICPrevScaledInput=0.0  OutMin=[]  OutMax=[]  OutDataType=fixdt(1, 16)  OutScaling=2^-10  DoSatur=off
  IIRgyroz : DiscreteFilter  Numerator=Estimator.IMU.filterGyroNum  Denominator=Estimator.IMU.filterGyroDen
  Logical Operator : Logic  Inputs=6  AllPortsSameDT=off  OutDataTypeStr=boolean
  Logical Operator1 : Logic  AllPortsSameDT=off  OutDataTypeStr=boolean
  Logical Operator2 : Logic  Operator=OR  AllPortsSameDT=off  OutDataTypeStr=boolean
  Logical Operator3 : Logic  Inputs=4  AllPortsSameDT=off  OutDataTypeStr=boolean
  Mux5 : Mux  Inputs=2
  Selectpitchroll : Selector  InputPortWidth=3  IndexOptions=Index vector (dialog)  Indices=[2 3]  OutputSizes=1
  maxdw1 : simulink/Logic and Bit Operations/Compare To Constant  relop=<=  const=Estimator.pos.ofDPQMax  OutDataTypeStr=boolean
  maxdw2 : simulink/Logic and Bit Operations/Compare To Constant  relop=<=  const=Estimator.pos.ofDPQMax  OutDataTypeStr=boolean
  maxp : simulink/Logic and Bit Operations/Compare To Constant  relop=<=  const=Estimator.pos.ofPitchRollMax  OutDataTypeStr=boolean
  maxp2 : simulink/Logic and Bit Operations/Compare To Constant  relop=<=  const=Estimator.pos.ofPQHovMax  OutDataTypeStr=boolean
  maxq : simulink/Logic and Bit Operations/Compare To Constant  relop=<=  const=Estimator.pos.ofPitchRollMax  OutDataTypeStr=boolean
  maxq2 : simulink/Logic and Bit Operations/Compare To Constant  relop=<=  const=Estimator.pos.ofPQHovMax  OutDataTypeStr=boolean
  maxw1 : simulink/Logic and Bit Operations/Compare To Constant  relop=<=  const=Estimator.pos.ofPQMax  OutDataTypeStr=boolean
  maxw2 : simulink/Logic and Bit Operations/Compare To Constant  relop=<=  const=Estimator.pos.ofPQMax  OutDataTypeStr=boolean
  maxw3 : simulink/Logic and Bit Operations/Compare To Constant  relop=<=  const=Estimator.pos.deltaDXYMax  OutDataTypeStr=boolean
  maxw4 : simulink/Logic and Bit Operations/Compare To Constant  relop=<=  const=Estimator.pos.deltaDXYMax  OutDataTypeStr=boolean
  minHeightforOF : simulink/Logic and Bit Operations/Compare To Constant  relop=<=  const=Estimator.pos.opticalFlowZMax  OutDataTypeStr=boolean
  enable_flag : Outport  VectorParamsAs1DForOutWhenUnconnected=off
  wires:
  minHeightforOF/1 -> Logical Operator3/4
  IIRgyroz/1 -> DiscreteDerivative/1
  Mux5/1 -> Demux1/1, Demux4/1, IIRgyroz/1
  maxw4/1 -> Logical Operator3/3
  maxw3/1 -> Logical Operator3/2
  dxyOF_datin/1 -> Add/1
  Demux3/2 -> Abs9/1
  Demux3/1 -> Abs8/1
  dxy_estimin/1 -> Add/2
  Add/1 -> Demux3/1
  Abs9/1 -> maxw4/1
  Abs8/1 -> maxw3/1
  Logical Operator2/1 -> Logical Operator3/1
  Logical Operator3/1 -> enable_flag/1
  DiscreteDerivative/1 -> Demux2/1  "dpq"
  Demux2/2 -> Abs7/1
  Demux2/1 -> Abs6/1
  Abs7/1 -> maxdw2/1
  Abs6/1 -> maxdw1/1
  Logical Operator1/1 -> Logical Operator2/2
  Demux1/2 -> Abs5/1
  Demux1/1 -> Abs4/1
  Abs5/1 -> maxq2/1
  Abs4/1 -> maxp2/1
  Abs3/1 -> maxq/1
  Abs2/1 -> maxp/1
  Demux4/2 -> Abs1/1
  Demux4/1 -> Abs/1
  Abs1/1 -> maxw2/1
  Abs/1 -> maxw1/1
  Z_estimin/1 -> minHeightforOF/1
  Logical Operator/1 -> Logical Operator2/1
  maxw1/1 -> Logical Operator/3
  Bus Selector/1 -> Mux5/1  "<p>"
  Selectpitchroll/1 -> Demux5/1
  sensorIMU_datin/1 -> Bus Selector/1
  maxq2/1 -> Logical Operator1/2
  Bus Selector/2 -> Mux5/2  "<q>"
  maxp/1 -> Logical Operator/1
  maxw2/1 -> Logical Operator/4
  orient_estimin/1 -> Selectpitchroll/1
  maxdw1/1 -> Logical Operator/5
  maxdw2/1 -> Logical Operator/6
  maxq/1 -> Logical Operator/2
  Demux5/1 -> Abs2/1
  Demux5/2 -> Abs3/1
  maxp2/1 -> Logical Operator1/1

== system flightControlSystem/Control System/State Estimator/XY Position Estimator/EstimatorVelocity/xy velocity w//o angular velocity compensation ==
  note: Optical flow raw readings are converted to velocity in m/s based on the estimated altitude
  optical_flow : Inport
  z_estimate : Inport  Port=2
  " " : Product  Inputs=**
  Compare To Constant : simulink/Logic and Bit Operations/Compare To Constant  relop=<  const=200*4  OutDataTypeStr=boolean
  Counter Free-Running : simulink/Sources/Counter Free-Running  NumBits=32  tsamp=-1
  Gain : Gain  Gain=-1
  Select dxy : Selector  InputPortWidth=3  IndexOptions=Index vector (dialog)  Indices=[1 2]  OutputSizes=1
  Switch : Switch  Criteria=u2 > Threshold  SaturateOnIntegerOverflow=off  InputSameDT=off
  opticalFlowErrorCorrect : Gain  Gain=1.15
  optical_flow_dx_dy : Outport
  wires:
  Select dxy/1 -> optical_flow_dx_dy/1  "optical_flow_dx_dy"
  " "/1 -> opticalFlowErrorCorrect/1
  opticalFlowErrorCorrect/1 -> Switch/3
  Gain/1 -> " "/2
  Switch/1 -> Select dxy/1
  Counter Free-Running/1 -> Compare To Constant/1
  Compare To Constant/1 -> Switch/2
  optical_flow/1 -> " "/1, Switch/1
  z_estimate/1 -> Gain/1

== matlab function flightControlSystem/Image Processing System/MATLAB Function ==
  data: bw input; n output; c output; area output; border output; ex output; ey output
function [n, c, area, border, ex, ey] = vision_features(bw)
    bw_mat = single(bw);
    [H, W] = size(bw_mat);
    
    r1 = floor(H/3);  r2 = floor(2*H/3);
    c1 = floor(W/3);  c2 = floor(2*W/3);
    
    n_fwd   = sum(sum(bw_mat(1:r1,    c1+1:c2)));
    n_right = sum(sum(bw_mat(r1+1:r2, c2+1:W)));
    n_back  = sum(sum(bw_mat(r2+1:H,  c1+1:c2)));
    n_left  = sum(sum(bw_mat(r1+1:r2, 1:c1)));
    n = single([n_fwd; n_right; n_back; n_left]);
    
    xs = single(1:W);  
    ys = single((1:H)');
    
    b_fwd = sum(bw_mat(1:r1,:), 1);       
    cF = sum(b_fwd.*xs)/max(sum(b_fwd),single(1)) - single(W/2);
    
    b_right = sum(bw_mat(:,c2+1:W), 2);   
    cR = single(H/2) - sum(b_right.*ys)/max(sum(b_right),single(1));
    
    b_back = sum(bw_mat(r2+1:H,:), 1);    
    cB = sum(b_back.*xs)/max(sum(b_back),single(1)) - single(W/2);
    
    b_left = sum(bw_mat(:,1:c1), 2);      
    cL = single(H/2) - sum(b_left.*ys)/max(sum(b_left),single(1));
    
    c = single([cF; cR; cB; cL]);
    area = single(sum(sum(bw_mat)));
    
    % --- thin 3-pixel border ring ---
    m = 3;
    border = single(sum(sum(bw_mat(1:m,:))) + sum(sum(bw_mat(H-m+1:H,:))) + ...
                    sum(sum(bw_mat(:,1:m))) + sum(sum(bw_mat(:,W-m+1:W))));
                    
    % --- centroid of the whole mask relative to image center ---
    tot = max(area, single(1));
    cx = sum(sum(bw_mat,1).*xs)/tot;
    cy = sum(sum(bw_mat,2).*ys)/tot;
    
    ex = single(cx - single(W/2));      
    ey = single(single(H/2) - cy);      
end

== matlab function flightControlSystem/Control System/Controller/Position Controller/Position error transformation (Earth to Body frame) ==
  data: yaw input; xy_err_earth input; xy_err_body output
function xy_err_body = fcn(yaw,xy_err_earth)

transformation = [cos(yaw), sin(yaw); -sin(yaw),  cos(yaw)];
xy_err_body = transformation * xy_err_earth;


end

== matlab function flightControlSystem/Control System/Path Planning/MATLAB Function ==
  data: yaw_est input; X_vel output; n input; c input; vision_flag input; Y_vel output; Yaw_cmd output; area input; Z_cmd output; border input; ex input; ey input
function [X_vel, Y_vel, Yaw_cmd, Z_cmd] = flight_logic(yaw_est, n, c, vision_flag, area, border, ex, ey)
    persistent locked_yaw mode prev_mode cnt integ land_cnt landing;
    
    if isempty(locked_yaw), locked_yaw = single(0); end
    if isempty(mode),       mode = single(1);       end
    if isempty(prev_mode),  prev_mode = single(0);  end
    if isempty(cnt),        cnt = single(0);        end
    if isempty(integ),      integ = single(0);      end
    if isempty(land_cnt),   land_cnt = single(0);   end
    if isempty(landing),    landing = false;        end

    Z_cmd   = single(-1.1);
    Yaw_cmd = single(locked_yaw); % Never rotate mid-flight
    
    if vision_flag <= 0
        X_vel = single(0); Y_vel = single(0); integ = single(0);
        locked_yaw = single(yaw_est); Yaw_cmd = single(yaw_est);
        return;
    end
    
    % ---------- LANDING: isolated blob fully inside the image = the circle ----------
    isCircle = (area > 150) && (border < 3);
    
    if isCircle || landing
        % P-control toward the circle centre (body frame: forward = ey, right = ex)
        Kc = single(0.004);
        vf = max(min(Kc*ey, single(0.10)), single(-0.10));
        vr = max(min(Kc*ex, single(0.10)), single(-0.10));
        
        if abs(ex) < 8 && abs(ey) < 8
            land_cnt = land_cnt + single(1);
        else
            land_cnt = single(0);
        end
        
        if land_cnt >= 3
            landing = true; % latch: never abort once committed
        end
        
        if landing
            Z_cmd = single(0);
            vf = single(0); vr = single(0);
        end
        
        X_vel = single((vf*cos(locked_yaw)) - (vr*sin(locked_yaw)));
        Y_vel = single((vf*sin(locked_yaw)) + (vr*cos(locked_yaw)));
        return;
    end
    
    % --- LINE FOLLOWING LOGIC ---
    D   = single([1 0; 0 1; -1 0; 0 -1]);
    THR = single(150);
    
    pA = single(mod(mode, 4) + 1);
    pB = single(mod(mode+2, 4) + 1);
    
    excl = single(0);
    if prev_mode > 0
        excl = single(mod(prev_mode+1, 4) + 1);
    end
    
    nA = n(pA); 
    nB = n(pB);
    if pA == excl, nA = single(0); end
    if pB == excl, nB = single(0); end
    
    side = max(nA, nB);
    
    if side > THR
        cnt = cnt + single(1);
    else
        cnt = single(0);
    end
    
    if cnt >= 2
        prev_mode = mode;
        if nA >= nB, mode = pA; else, mode = pB; end
        cnt = single(0); integ = single(0);
    end
    
    v = single(0.12);
    if side > THR/4, v = single(0.05); end
    
    e = c(mode);
    
    if n(mode) < single(15)
        corr = single(0);          
        v = single(0.08);          
        integ = single(0);         
    else
        integ = integ + e;
        if integ > 300, integ = single(300);
        elseif integ < -300, integ = single(-300); end
        
        corr = (single(0.002) * e) + (single(0.00005) * integ);
        
        if corr > 0.15, corr = single(0.15);
        elseif corr < -0.15, corr = single(-0.15); end
    end
    
    if mod(mode, 2) == 1
        ax = single([0; 1]); 
    else
        ax = single([1; 0]); 
    end
    
    v_body_1 = (v * D(mode, 1)) + (corr * ax(1));
    v_body_2 = (v * D(mode, 2)) + (corr * ax(2));
    
    X_vel = single((v_body_1 * cos(locked_yaw)) - (v_body_2 * sin(locked_yaw)));
    Y_vel = single((v_body_1 * sin(locked_yaw)) + (v_body_2 * cos(locked_yaw)));
end
